simulink model "Guardian_Battery_for_integrated"  (R2025b)
settings: Solver=FixedStepDiscrete  StartTime=0.0  StopTime=T_end_s  FixedStep=0.1  RelTol=1e-3
values from neighbouring files (symbols this model uses):
  a1_coef = exp(-Ts/(tau1_s))    [Integrated_Project_Script.m]
  a2_coef = exp(-Ts/(tau2_s))    [Integrated_Project_Script.m]
  Q_nominal = 50    [Integrated_Project_Script.m]
  R0_ref = 0.0007    [Integrated_Project_Script.m]
  R1_ref = 0.0016    [Integrated_Project_Script.m]
  R2_ref = 0.00035    [Integrated_Project_Script.m]
  Ts_hyst_ref = 1    [Integrated_Project_Script.m]
undefined symbols (not defined in the file or in its folder): DiscIntNeverNeededParam, dspblkCoreblockFVToolHelper, gcbh
libraries: simulink x3
settings Model: Creator=LENOVO  LastModifiedBy=LENOVO

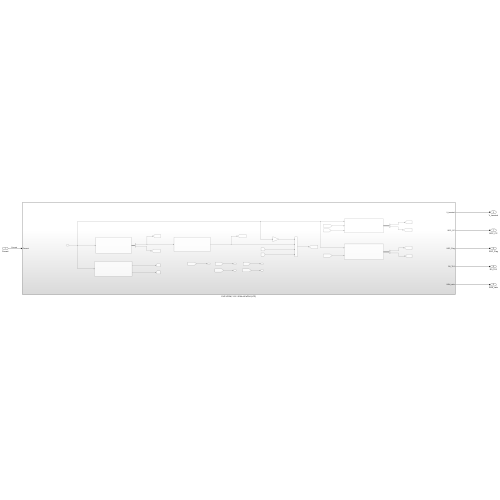
[thumbnail: Simulink's stored preview of the top-level diagram]
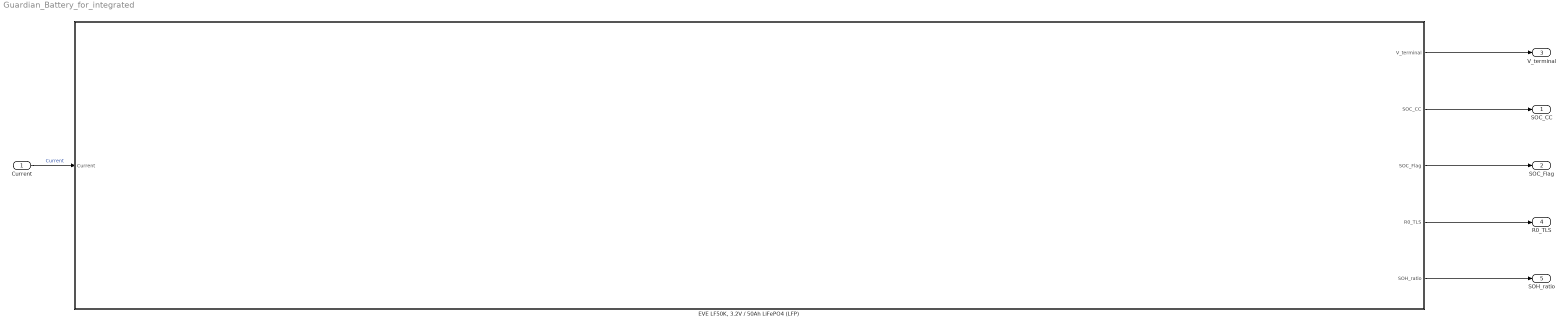
== system Guardian_Battery_for_integrated ==
  Current : Inport
  "EVE LF50K, 3.2V / 50Ah LiFePO4 (LFP)" : Subsystem
  SOC_CC : Outport
  SOC_Flag : Outport  Port=2
  V_terminal : Outport  Port=3
  R0_TLS : Outport  Port=4
  SOH_ratio : Outport  Port=5
  wires:
  Current/1 -> "EVE LF50K, 3.2V / 50Ah LiFePO4 (LFP)"/1(Current)  "Current"
  "EVE LF50K, 3.2V / 50Ah LiFePO4 (LFP)"/1(V_terminal) -> V_terminal/1
  "EVE LF50K, 3.2V / 50Ah LiFePO4 (LFP)"/2(SOC_CC) -> SOC_CC/1
  "EVE LF50K, 3.2V / 50Ah LiFePO4 (LFP)"/3(SOC_Flag) -> SOC_Flag/1
  "EVE LF50K, 3.2V / 50Ah LiFePO4 (LFP)"/4(R0_TLS) -> R0_TLS/1
  "EVE LF50K, 3.2V / 50Ah LiFePO4 (LFP)"/5(SOH_ratio) -> SOH_ratio/1

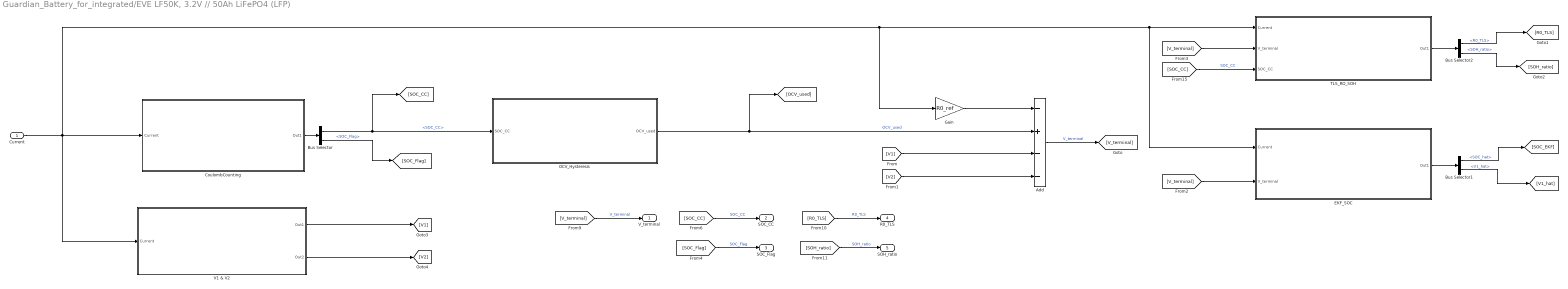
== system Guardian_Battery_for_integrated/EVE LF50K, 3.2V // 50Ah LiFePO4 (LFP) ==
  Current : Inport
  Add : Sum  Inputs=-+--
  Bus Selector : BusSelector  OutputSignals=SOC_CC,SOC_Flag
  Bus Selector1 : BusSelector  OutputSignals=SOC_hat,V1_hat
  Bus Selector2 : BusSelector  OutputSignals=R0_TLS,SOH_ratio
  CoulombCounting : Subsystem
  EKF_SOC : Subsystem
  Gain : Gain  Gain=R0_ref
  OCV_Hysteresis : Subsystem
  TLS_RO_SOH : Subsystem
  V1 & V2 : Subsystem
  V_terminal : Outport
  SOC_CC : Outport  Port=2
  SOC_Flag : Outport  Port=3
  R0_TLS : Outport  Port=4
  SOH_ratio : Outport  Port=5
  wires:
  V1 & V2/1(Out1) -> [V1]
  CoulombCounting/1(Out1) -> Bus Selector/1
  Bus Selector/2 -> [SOC_Flag]  "<SOC_Flag>"
  V1 & V2/2(Out2) -> [V2]
  Bus Selector/1 -> [SOC_CC], OCV_Hysteresis/1(SOC_CC)  "<SOC_CC>"
  OCV_Hysteresis/1(OCV_used) -> Add/2, [OCV_used]  "OCV_used"
  Current/1 -> TLS_RO_SOH/1(Current), EKF_SOC/1(Current), Gain/1, CoulombCounting/1(Current), V1 & V2/1(Current)
  Add/1 -> [V_terminal]  "V_terminal"
  Gain/1 -> Add/1
  [V1] -> Add/3
  [V2] -> Add/4
  [SOC_CC] -> TLS_RO_SOH/3(SOC_CC)  "SOC_CC"
  Bus Selector1/1 -> [SOC_EKF]  "<SOC_hat>"
  EKF_SOC/1(Out1) -> Bus Selector1/1
  Bus Selector1/2 -> [V1_hat]  "<V1_hat>"
  Bus Selector2/2 -> [SOH_ratio]  "<SOH_ratio>"
  Bus Selector2/1 -> [R0_TLS]  "<R0_TLS>"
  TLS_RO_SOH/1(Out1) -> Bus Selector2/1
  [V_terminal] -> TLS_RO_SOH/2(V_terminal)
  [V_terminal] -> EKF_SOC/2(V_terminal)
  [SOC_CC] -> SOC_CC/1  "SOC_CC"
  [SOC_Flag] -> SOC_Flag/1  "SOC_Flag"
  [V_terminal] -> V_terminal/1  "V_terminal"
  [R0_TLS] -> R0_TLS/1  "R0_TLS"
  [SOH_ratio] -> SOH_ratio/1  "SOH_ratio"

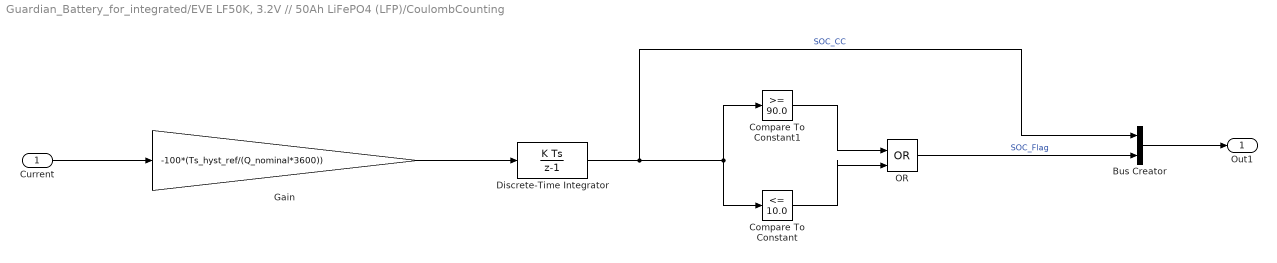
== system Guardian_Battery_for_integrated/EVE LF50K, 3.2V // 50Ah LiFePO4 (LFP)/CoulombCounting ==
  Current : Inport
  Bus Creator : BusCreator  Inputs=2
  Compare To Constant : simulink/Logic and Bit Operations/Compare To Constant  relop=<=  const=10.0  OutDataTypeStr=boolean
  Compare To Constant1 : simulink/Logic and Bit Operations/Compare To Constant  relop=>=  const=90.0  OutDataTypeStr=boolean
  Discrete-Time Integrator : DiscreteIntegrator  InitialCondition=80  SampleTime=-1  LimitOutput=on  UpperSaturationLimit=90  LowerSaturationLimit=10  ICPrevOutput=DiscIntNeverNeededParam  ICPrevScaledInput=DiscIntNeverNeededParam
  Gain : Gain  Gain=-100*(Ts_hyst_ref/(Q_nominal*3600))
  OR : Logic  Operator=OR  IconShape=distinctive  AllPortsSameDT=off  OutDataTypeStr=boolean
  Out1 : Outport
  wires:
  Current/1 -> Gain/1
  Gain/1 -> Discrete-Time Integrator/1
  Discrete-Time Integrator/1 -> Bus Creator/1, Compare To Constant1/1, Compare To Constant/1  "SOC_CC"
  Compare To Constant1/1 -> OR/1
  Compare To Constant/1 -> OR/2
  OR/1 -> Bus Creator/2  "SOC_Flag"
  Bus Creator/1 -> Out1/1

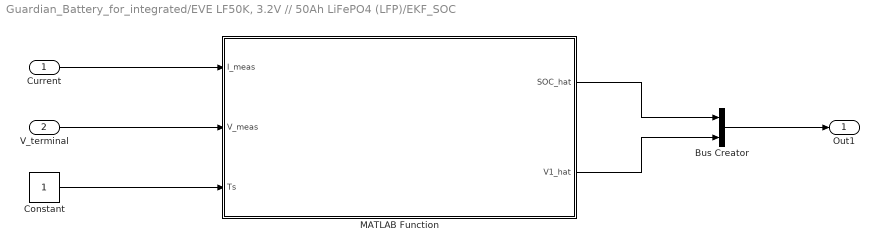
== system Guardian_Battery_for_integrated/EVE LF50K, 3.2V // 50Ah LiFePO4 (LFP)/EKF_SOC ==
  Current : Inport
  V_terminal : Inport  Port=2
  Bus Creator : BusCreator  Inputs=2
  Constant : Constant
  MATLAB Function : MATLAB Function  TreatAsAtomicUnit=on
  Out1 : Outport
  wires:
  Current/1 -> MATLAB Function/1(I_meas)
  V_terminal/1 -> MATLAB Function/2(V_meas)
  Constant/1 -> MATLAB Function/3(Ts)
  MATLAB Function/1(SOC_hat) -> Bus Creator/1
  MATLAB Function/2(V1_hat) -> Bus Creator/2
  Bus Creator/1 -> Out1/1

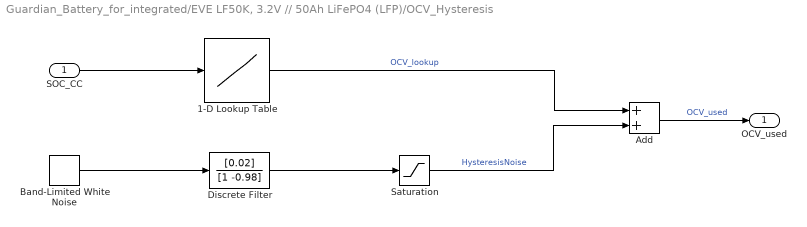
== system Guardian_Battery_for_integrated/EVE LF50K, 3.2V // 50Ah LiFePO4 (LFP)/OCV_Hysteresis ==
  SOC_CC : Inport
  1-D Lookup Table : Lookup_n-D  NumberOfTableDimensions=1  BreakpointsForDimension1=[0 5 10 20 30 40 50 60 70 80 90 95 100]  Table=[2.5 2.95 3.05 3.15 3.2 3.22 3.24 3.26 3.28 3.3 3.33 3.45 3.65]  ExtrapMethod=Clip  InternalRulePriority=Speed  RndMeth=Simplest
  Add : Sum
  Band-Limited White Noise : simulink/Sources/Band-Limited White Noise  Cov=[1e-4]  Ts=1  seed=[23341]
  Discrete Filter : DiscreteFilter  LoadFcn=dspblkCoreblockFVToolHelper(gcbh,'load');  Numerator=[0.02]  Denominator=[1 -0.98]
      settings: CopyFcn=dspblkCoreblockFVToolHelper(gcbh,'copy');  DeleteFcn=dspblkCoreblockFVToolHelper(gcbh,'close');  ModelCloseFcn=dspblkCoreblockFVToolHelper(gcbh,'close');  PreSaveFcn=dspblkCoreblockFVToolHelper(gcbh,'presave');  PostSaveFcn=dspblkCoreblockFVToolHelper(gcbh,'postsave');  CloseFcn=dspblkCoreblockFVToolHelper(gcbh,'close');
  Saturation : Saturate  UpperLimit=0.005  LowerLimit=-0.005
  OCV_used : Outport
  wires:
  SOC_CC/1 -> 1-D Lookup Table/1
  1-D Lookup Table/1 -> Add/1  "OCV_lookup"
  Band-Limited White Noise/1 -> Discrete Filter/1
  Discrete Filter/1 -> Saturation/1
  Saturation/1 -> Add/2  "HysteresisNoise"
  Add/1 -> OCV_used/1  "OCV_used"

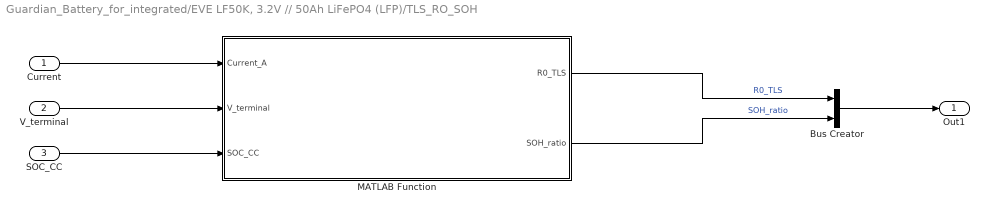
== system Guardian_Battery_for_integrated/EVE LF50K, 3.2V // 50Ah LiFePO4 (LFP)/TLS_RO_SOH ==
  Current : Inport
  V_terminal : Inport  Port=2
  SOC_CC : Inport  Port=3
  Bus Creator : BusCreator  Inputs=2
  MATLAB Function : MATLAB Function  TreatAsAtomicUnit=on
  Out1 : Outport
  wires:
  Current/1 -> MATLAB Function/1(Current_A)
  V_terminal/1 -> MATLAB Function/2(V_terminal)
  SOC_CC/1 -> MATLAB Function/3(SOC_CC)
  MATLAB Function/1(R0_TLS) -> Bus Creator/1  "R0_TLS"
  MATLAB Function/2(SOH_ratio) -> Bus Creator/2  "SOH_ratio"
  Bus Creator/1 -> Out1/1

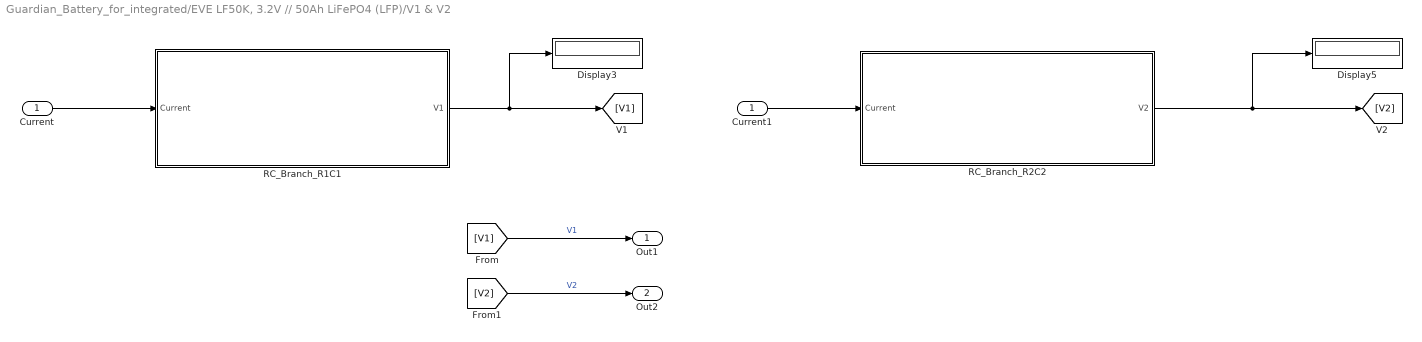
== system Guardian_Battery_for_integrated/EVE LF50K, 3.2V // 50Ah LiFePO4 (LFP)/V1 & V2 ==
  Current : Inport
  Current1 : InportShadow
  Display3 : Display
  Display5 : Display
  RC_Branch_R1C1 : Subsystem
  RC_Branch_R2C2 : Subsystem
  Out1 : Outport
  Out2 : Outport  Port=2
  wires:
  Current1/1 -> RC_Branch_R2C2/1(Current)
  RC_Branch_R1C1/1(V1) -> [V1], Display3/1
  Current/1 -> RC_Branch_R1C1/1(Current)
  RC_Branch_R2C2/1(V2) -> [V2], Display5/1
  [V1] -> Out1/1  "V1"
  [V2] -> Out2/1  "V2"

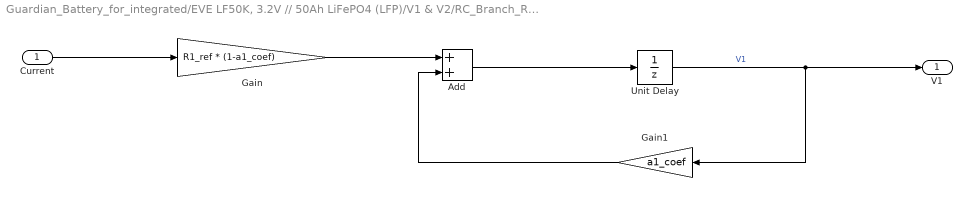
== system Guardian_Battery_for_integrated/EVE LF50K, 3.2V // 50Ah LiFePO4 (LFP)/V1 & V2/RC_Branch_R1C1 ==
  Current : Inport
  Add : Sum
  Gain : Gain  Gain=R1_ref * (1-a1_coef)
  Gain1 : Gain  Gain=a1_coef
  Unit Delay : UnitDelay  SampleTime=-1  HasFrameUpgradeWarning=on
  V1 : Outport
  wires:
  Current/1 -> Gain/1
  Gain/1 -> Add/1
  Add/1 -> Unit Delay/1
  Unit Delay/1 -> Gain1/1, V1/1  "V1"
  Gain1/1 -> Add/2

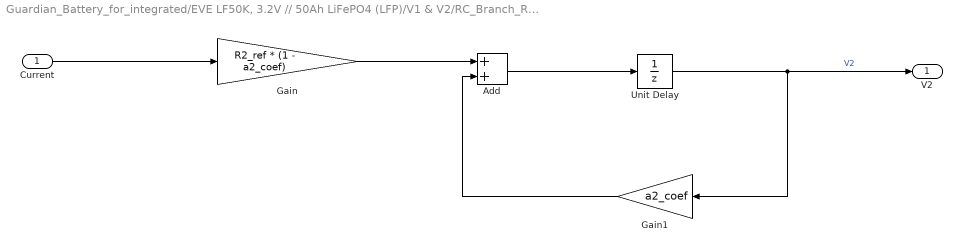
== system Guardian_Battery_for_integrated/EVE LF50K, 3.2V // 50Ah LiFePO4 (LFP)/V1 & V2/RC_Branch_R2C2 ==
  Current : Inport
  Add : Sum
  Gain : Gain  Gain=R2_ref * (1 - a2_coef)
  Gain1 : Gain  Gain=a2_coef
  Unit Delay : UnitDelay  SampleTime=-1  HasFrameUpgradeWarning=on
  V2 : Outport
  wires:
  Current/1 -> Gain/1
  Gain/1 -> Add/1
  Add/1 -> Unit Delay/1
  Unit Delay/1 -> Gain1/1, V2/1  "V2"
  Gain1/1 -> Add/2

== matlab function Guardian_Battery_for_integrated/EVE LF50K, 3.2V // 50Ah LiFePO4 (LFP)/TLS_RO_SOH/MATLAB Function ==
  data: Current_A input; R0_TLS output; V_terminal input; SOC_CC input; SOH_ratio output
function [R0_TLS, SOH_ratio] = TLS_RO_SOH_block(Current_A, V_terminal, SOC_CC)

R0 = 0.0007; % ohm
R1 = 0.0016; % ohm
C1 = 17000; % F
soc_bp = [0 5 10 20 30 40 50 60 70 80 90 95 100];
ocv_bp = [2.50 2.95 3.05 3.15 3.20 3.22 3.24 3.26 3.28 3.30 3.33 3.45 3.65];

%#codegen
% Bonus 3 - TLS-based R0 identification + SOH ratio (Sec. 6.5 / Figure 4)
%
% WIRING (inside the existing empty TLS_RO_SOH_Subsystem, SID 123):
%   In1 -> Current_A     (A,  from Current_A source)
%   In2 -> V_terminal     (V,  from logged Terminal_Voltage)
%   In3 -> SOC_CC          (%,  from logged SOC_CC)
%   Out1 -> R0_TLS (ohm)   -- ADD a second Outport, Out2 -> SOH_ratio (%)
%
% PARAMETERS (add via the block's Symbols/Editor pane as PARAMETERS,
% not Inputs, so they resolve from the base workspace exactly like the
% Gain/Lookup blocks elsewhere in this model -- do not hardcode numbers):
%   R1, C1        -> same R1, C1 already defined in Guardian_Battery_script.m
%   R0             -> the datasheet R0 (0.0007 ohm) from the same script
%   soc_bp, ocv_bp -> the OCV-SOC breakpoints already loaded from
%                      Guardian_Battery_OCV_SOC_Table.csv

persistent x_buf y_buf V1_hat n k R0_TLS_hold SOH_ratio_hold

Ts = 1; % s, matches the dataset's native rate (Sec. 3.2)

if isempty(k)
    n = 3600;               % drive-cycle length (Sec. 10: 3600 points at 1 Hz)
    x_buf = zeros(n,1);
    y_buf = zeros(n,1);
    V1_hat = 0;              % V1_hat(0): battery assumed at rest, no polarization
    k = 0;
    R0_TLS_hold = 0;
    SOH_ratio_hold = 0;
end

a1 = exp(-Ts/(R1*C1));

k = k + 1;
if k > n
    k = n;
end

% --- Figure 4, box 3: target y(k) and regressor x(k) ---------------------
% NOTE: uses V1_hat(k), i.e. the value BEFORE this step's update, to match
% the index convention in Sec. 6.5:
%   y(k) = OCV_used(SOC_CC(k)) - V1_hat(k) - V_meas(k)
%   x(k) = I(k)
OCV_k = interp1(soc_bp, ocv_bp, SOC_CC, 'linear', 'extrap');
y_buf(k) = OCV_k - V1_hat - V_terminal;
x_buf(k) = Current_A;

% --- Figure 4, box 2: THEN advance V1_hat open-loop, given R1,C1 ---------
V1_hat = a1*V1_hat + R1*(1-a1)*Current_A;

% --- Figure 4, boxes 4-6: run once, on the final sample -------------------
if k == n
    x = x_buf - mean(x_buf);
    y = y_buf - mean(y_buf);
    D = [x, y];
    [~, ~, V] = svd(D, 0);
    R0_TLS_hold  = -V(1,2) / V(2,2);
    SOH_ratio_hold = (R0 / R0_TLS_hold) * 100;
end

R0_TLS    = R0_TLS_hold;
SOH_ratio = SOH_ratio_hold;

== matlab function Guardian_Battery_for_integrated/EVE LF50K, 3.2V // 50Ah LiFePO4 (LFP)/EKF_SOC/MATLAB Function ==
  data: I_meas input; SOC_hat output; V_meas input; Ts input; V1_hat output
function [SOC_hat, V1_hat] = EKF_SOC_Estimator(I_meas, V_meas, Ts)
%EKF_SOC_ESTIMATOR  Extended Kalman Filter SOC estimator for the Guardian
%   Battery ECM Project (1RC Thevenin model, LF50K 3.2V/50Ah LFP cell).
%
%   [SOC_hat, V1_hat] = EKF_SOC_Estimator(I_meas, V_meas, Ts)
%
%   Inputs:
%     I_meas  - measured cell current (A), discharge = POSITIVE
%     V_meas  - measured terminal voltage (V)
%     Ts      - sample time (s) -- must match the model's discrete step
%
%   Outputs:
%     SOC_hat - estimated state of charge (%)
%     V1_hat  - estimated RC-branch polarization voltage (V)
%
%   THIS FILE IS PROVIDED AS-IS. Do not modify the cell parameters,
%   OCV breakpoints, or filter structure -- only the noise tuning
%   (Qcov, Rcov) and initial covariance (P0) are meant to be adjusted
%   by students, and only if they can justify the change in their report.
%
%   Usage in Simulink: paste this exact function body into a MATLAB
%   Function block with two inputs (I_meas, V_meas) and two outputs
%   (SOC_hat, V1_hat). Pass Ts as a block mask parameter or hardcode it
%   to match your model's Fixed-Step discrete sample time.
%
%   Guardian Battery ECM Project - Part 2 Addendum
%   Reference cell parameters: see project datasheet, Appendix A.

%#codegen
persistent x P initialized
if isempty(initialized)
    x = [80; 0];            % initial state estimate [SOC(%); V1(V)]
                             % (80% matches the shared drive-cycle test's
                             % given initial condition -- do not change
                             % unless your report explains a cold-start
                             % scenario with an unknown initial SOC)
    P = diag([4, 0.01]);    % initial covariance
    initialized = true;
end

% ---- Fixed cell/model parameters (from project datasheet, Appendix A) ----
Q_nominal_Ah = 50;
R0 = 0.00070;      % ohm  (datasheet AC impedance, 1 kHz, mid-SOC, 25 C)
R1 = 0.00160;      % ohm  (scaled from literature HPPC fit, see Appendix A)
C1 = 17000;        % F
tau1 = R1 * C1;
a = exp(-Ts / tau1);

% ---- OCV-SOC breakpoints -- MUST match Guardian_Battery_OCV_SOC_Table.csv ----
soc_bp = [0 5 10 20 30 40 50 60 70 80 90 95 100];
ocv_bp = [2.50 2.95 3.05 3.15 3.20 3.22 3.24 3.26 3.28 3.30 3.33 3.45 3.65];

% ---- Process/measurement noise tuning ----
% Qcov reflects trust in the process model (SOC integration, V1 dynamics).
% Rcov reflects trust in the voltage measurement (~20 mV sensor noise assumed).
% Students may retune these two lines; document any change and why.
Qcov = diag([1e-3, 1e-6]);
Rcov = 4e-4;

% =====================================================================
% PREDICT
% =====================================================================
SOC_pred = x(1) - (Ts / (Q_nominal_Ah * 3600)) * I_meas * 100;
V1_pred  = a * x(2) + R1 * (1 - a) * I_meas;
x_pred = [SOC_pred; V1_pred];

F = [1, 0; 0, a];
P_pred = F * P * F' + Qcov;

% =====================================================================
% UPDATE
% =====================================================================
OCV_pred  = interp1(soc_bp, ocv_bp, x_pred(1), 'linear', 'extrap');

% Local OCV slope (finite-difference approximation of dOCV/dSOC at the
% predicted operating point) -- this is the nonlinear part of the EKF;
% a standard Kalman filter cannot handle this curved OCV(SOC) relationship.
d = 0.5;
dOCV_dSOC = interp1(soc_bp, ocv_bp, x_pred(1) + d, 'linear', 'extrap') ...
          - interp1(soc_bp, ocv_bp, x_pred(1) - d, 'linear', 'extrap');
dOCV_dSOC = dOCV_dSOC / (2 * d);

H = [dOCV_dSOC, -1];

V_pred = OCV_pred - I_meas * R0 - x_pred(2);
y_resid = V_meas - V_pred;

S = H * P_pred * H' + Rcov;
K = P_pred * H' / S;

x = x_pred + K * y_resid;
P = (eye(2) - K * H) * P_pred;

% Physical bound -- SOC cannot leave [0, 100]%
x(1) = min(max(x(1), 0), 100);

SOC_hat = x(1);
V1_hat  = x(2);

end
